simulink model "drive_side"  (R2026b)
settings: Solver=VariableStepAuto
model mask{side=1}
  mask prompts: side "Side (1 = Left / node 1, 2 = Right / node 2)"
undefined symbols (not defined in the file or in its folder): DiscIntNeverNeededParam, P
libraries: simulink x1
settings Model: Creator=aomar  LastModifiedBy=aomar

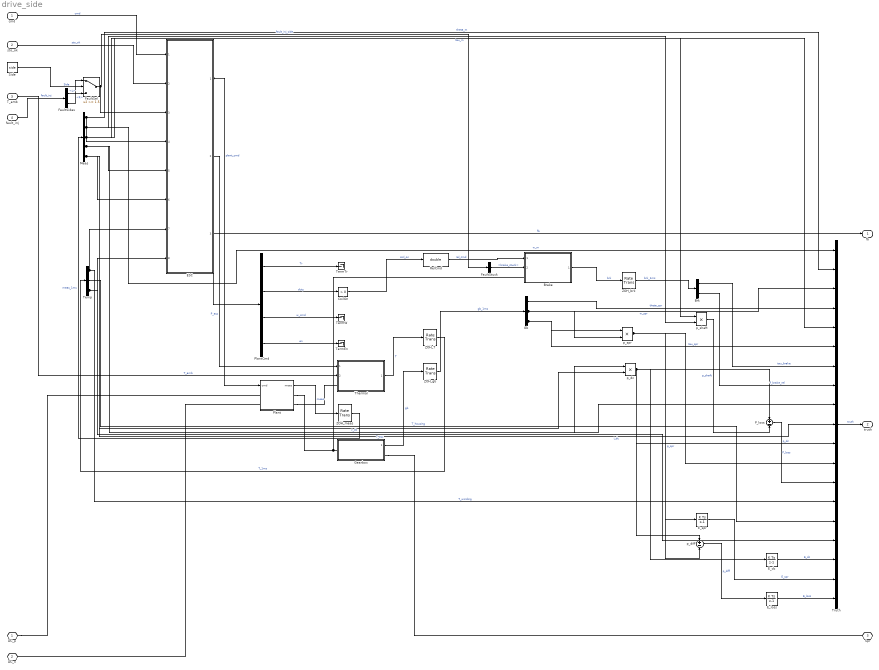
== system drive_side ==
  cmd : Inport  OutDataTypeStr=Bus: Bus_DriveSideCmd  SampleTime=P.drive.Ts_esc
  sto_ok : Inport  Port=2  OutDataTypeStr=boolean  SampleTime=P.drive.Ts_esc
  T_amb : Inport  Port=3  OutDataTypeStr=double  SampleTime=P.drive.Ts_esc
  fault_inj : Inport  Port=4  OutDataTypeStr=Bus: Bus_DriveFaultInj  SampleTime=P.drive.Ts_esc
  Brake : Subsystem  ReferencedSubsystem=drive_brake
  Brk : Demux  Outputs=2
  CoilOn : simulink/Logic and Bit Operations/Compare To Constant  relop=>  const=0  OutDataTypeStr=boolean
  ESC : Subsystem  ReferencedSubsystem=drive_esc
  E_dc : DiscreteIntegrator  gainval=1  SampleTime=P.drive.Ts_esc  ICPrevOutput=DiscIntNeverNeededParam  ICPrevScaledInput=DiscIntNeverNeededParam
  E_loss : DiscreteIntegrator  gainval=1  SampleTime=P.drive.Ts_esc  ICPrevOutput=DiscIntNeverNeededParam  ICPrevScaledInput=DiscIntNeverNeededParam
  E_spr : DiscreteIntegrator  gainval=1  SampleTime=P.drive.Ts_esc  ICPrevOutput=DiscIntNeverNeededParam  ICPrevScaledInput=DiscIntNeverNeededParam
  FaultSel : Switch  Threshold=1.5  SaturateOnIntegerOverflow=off  InputSameDT=off
  FaultSides : BusSelector  OutputSignals=L,R
  FaultStuck : BusSelector  OutputSignals=brake_stuck
  Gb : Demux  Outputs=3
  Gearbox : Subsystem  ReferencedSubsystem=drive_gearbox
  Meas : Demux  Outputs=5
  P_loss : Sum  Inputs=+-
  Plant : Subsystem  Variant=on
  PlantCmd : Demux
  RelCmd : DataTypeConversion  OutDataTypeStr=double  RndMeth=Nearest
  Side : Constant  Value=side
  Temp : Demux  Outputs=3
  TermEn : Terminator
  TermTr : Terminator
  TermW : Terminator
  Thermal : Subsystem  ReferencedSubsystem=drive_thermal
  Truth : BusCreator  Inputs=19  OutDataTypeStr=Bus: Bus_DriveSideTruth  NonVirtualBus=on
  ZOH_T : RateTransition  OutPortSampleTime=P.drive.Ts_esc
  ZOH_brk : RateTransition  OutPortSampleTime=P.drive.Ts_esc
  ZOH_gb : RateTransition  OutPortSampleTime=P.drive.Ts_esc
  ZOH_meas : RateTransition  OutPortSampleTime=P.drive.Ts_esc
  p_dc : Product  Inputs=**
  p_diff : Sum  Inputs=+-
  p_shaft : Product  Inputs=**
  p_spr : Product  Inputs=**
  DC_p : PMIOPort  Side=Left  ConnectionType=Connection: foundation.electrical.electrical
  DC_n : PMIOPort  Port=2  Side=Left  ConnectionType=Connection: foundation.electrical.electrical
  Spr : PMIOPort  Port=3  Side=Right  ConnectionType=Connection: foundation.mechanical.rotational.rotational
  fb : Outport  OutDataTypeStr=Bus: Bus_DriveSideFb
  truth : Outport  Port=2  OutDataTypeStr=Bus: Bus_DriveSideTruth
  wires:
  cmd/1 -> ESC/1  "cmd"
  sto_ok/1 -> ESC/2  "sto_ok"
  Side/1 -> FaultSel/2  "Side"
  T_amb/1 -> Thermal/2  "T_amb"
  fault_inj/1 -> FaultSides/1  "fault_inj"
  FaultSides/1 -> FaultSel/3  "<L>"
  FaultSides/2 -> FaultSel/1  "<R>"
  Meas/1 -> Truth/2, ESC/4  "theta_m"
  Meas/2 -> p_shaft/2, Truth/1  "w_m"
  Meas/3 -> Truth/5, p_shaft/1  "tau_m"
  Meas/4 -> Truth/9, p_dc/1, ESC/5  "v_dc"
  Meas/5 -> Truth/10, p_dc/2, ESC/6  "i_dc"
  Temp/1 -> Truth/14, ESC/7  "T_winding"
  Temp/2 -> Truth/15  "T_housing"
  Temp/3 -> Truth/16, ESC/8  "T_esc"
  FaultSel/1 -> FaultStuck/1, ESC/3  "fault_inj_side"
  ESC/1 -> Plant/1(cmd), PlantCmd/1  "plant_cmd"
  ESC/2 -> Thermal/1  "P_esc"
  ESC/3 -> fb/1  "fb"
  PlantCmd/1 -> TermTr/1  "Tr"
  PlantCmd/2 -> CoilOn/1  "duty"
  PlantCmd/3 -> TermW/1  "w_cmd"
  PlantCmd/4 -> TermEn/1  "en"
  Plant/1(meas) -> ZOH_meas/1  "meas"
  CoilOn/1 -> RelCmd/1  "coil_on"
  ZOH_meas/1 -> Meas/1  "meas_1ms"
  Thermal/1 -> ZOH_T/1  "T"
  Gearbox/1 -> ZOH_gb/1  "gb"
  ZOH_T/1 -> Temp/1  "T_1ms"
  ZOH_gb/1 -> Gb/1  "gb_1ms"
  RelCmd/1 -> Brake/1  "rel_cmd"
  FaultStuck/1 -> Brake/2  "<brake_stuck>"
  Gb/1 -> Truth/4  "theta_spr"
  Gb/2 -> p_spr/2, Truth/3  "w_spr"
  Gb/3 -> Truth/6, p_spr/1  "tau_spr"
  Brake/1 -> ZOH_brk/1  "brk"
  p_spr/1 -> p_diff/2, E_spr/1, Truth/12  "p_spr"
  ZOH_brk/1 -> Brk/1  "brk_1ms"
  p_dc/1 -> E_dc/1, p_diff/1, Truth/11, P_loss/1  "p_dc"
  Brk/1 -> Truth/7  "tau_brake"
  Brk/2 -> Truth/8  "f_brake_rel"
  p_diff/1 -> E_loss/1  "p_diff"
  p_shaft/1 -> P_loss/2  "p_shaft"
  E_spr/1 -> Truth/18  "E_spr"
  P_loss/1 -> Truth/13  "P_loss"
  E_dc/1 -> Truth/17  "E_dc"
  E_loss/1 -> Truth/19  "E_loss"
  Truth/1 -> truth/1  "truth"
  connections:
  Gearbox/LConn1 -- Plant/RConn1 -- Brake/LConn1
  Plant/LConn2 -- DC_n/RConn1
  DC_p/RConn1 -- Plant/LConn1
  Gearbox/RConn1 -- Spr/RConn1
  Plant/RConn2 -- Thermal/LConn1

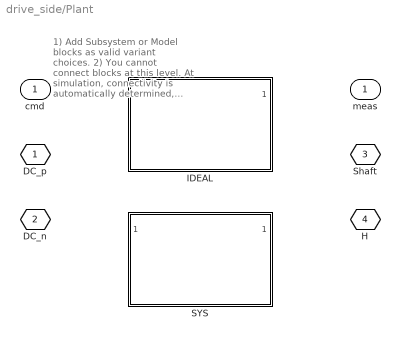
== system drive_side/Plant ==
  note: 1) Add Subsystem or Model blocks as valid variant choices.
      | 2) You cannot connect blocks at this level. At simulation, connectivity is automatically
      | determined, based on the active variant and port name matching.
  cmd : Inport
  IDEAL : Subsystem  VariantControl=VC_DRIVE_FID == 3  ReferencedSubsystem=drive_plant_ideal
  SYS : Subsystem  VariantControl=VC_DRIVE_FID == 1  ReferencedSubsystem=drive_plant_sys
  DC_p : PMIOPort  Side=Left  ConnectionType=Connection: foundation.electrical.electrical
  DC_n : PMIOPort  Port=2  Side=Left  ConnectionType=Connection: foundation.electrical.electrical
  Shaft : PMIOPort  Port=3  Side=Right  ConnectionType=Connection: foundation.mechanical.rotational.rotational
  H : PMIOPort  Port=4  Side=Right  ConnectionType=Connection: foundation.thermal.thermal
  meas : Outport
